simulink model "pmsm_foc_model"  (R2024b)
settings: Solver=ode4  StartTime=0.0  StopTime=.25001  FixedStep=5e-6  RelTol=1e-3
InitFcn:
  | model_dir=fileparts(get_param(bdroot,'FileName')); addpath(fullfile(model_dir,'..','matlab')); addpath(fullfile(model_dir,'..','..','..','build','research_host'));
model workspace (MAT data in the model file):
  cfg.p.Rs = 5.5
  cfg.p.Ld = 0.0007185
  cfg.p.Lq = 0.000905
  cfg.p.psi = 0.00257
  cfg.p.poles = 7
  cfg.p.Vbus = 12
  cfg.p.shunt = 0.02
  cfg.p.gain = 50
  cfg.p.Vref = 3.3
  cfg.p.bits = 12
  cfg.p.ref = 1.65
  cfg.p.lsb = 0.0008056640625
  cfg.p.Ts = 0.001
  cfg.p.fpwm = 20000
  cfg.p.adc_clock = 12000000
  cfg.p.aperture = 6.25e-07
  cfg.p.conversion = 1.66666666667e-06
  cfg.p.bw = 80000
  cfg.p.recovery_tau = 2e-05
  cfg.p.b0 = [0.004 -0.003]
  cfg.p.k = [0.123 0.118]
  cfg.p.kp = 0.5
  cfg.p.ki = 150
  cfg.p.tracking = 200
  cfg.p.ref_limit = 0.04
  cfg.p.mod_limit = 0.0577350269
  cfg.p.seed = 2801
  cfg.dt = 5e-06
  cfg.duration = 0.25
  cfg.reference = 0.04
  cfg.method = "offline_M1"
  cfg.guard = "original"
  cfg.bias_model = "M1"
  cfg.sensor_noise = 0.0008
  cfg.seed = 2801
  cfg.delay = 0.000775
  cfg.omega = 0
  cfg.motion = "locked"
  cfg.J = 2e-05
  cfg.B = 2e-05
  cfg.load = 0
  cfg.adc_phase_s = 0.00025
  cfg.Rfactor = 1
  cfg.Lfactor = 1
  cfg.psifactor = 1
  cfg.bus = 12
  cfg.bias_factor = 1
  cfg.temp_shift = 0
  cfg.esoA = [0.00114141670648  0; 0  1]
  cfg.esoB = [0.181610651508; 0]
  cfg.esoC = [1 1]
  cfg.esoK = [-663.509924553; 0.016548610477]
  cfg.certified = 0
  cfg.error_bound = [0.003; 0.003]
  cfg.fit.model = "M1"
  cfg.fit.coef = {[0.00396479988498; 0.123043689108], [-0.00296998501666; 0.117863719572]}
  cfg.fit.ci95 = {[0.00382515493307  0.00410444483689; 0.122781063704  0.123306314513], [-0.00311154324492  -0.00282842678841; 0.117594560495  0.118132878649]}
  cfg.fit.rank = [2 2]
  cfg.fit.condition = [7.72107695202 7.575631139]
  cfg.noise = [3.05609968406e-05 0.000138698185568 -0.00168675785383 -0.00117877986568 0.000708300191208 0.000612576864667 0.000162588627627 0.000618469759852 0.00109376547218 -0.00161987518611 -0.00119761794175 -0.000644839674806 ... (504 elements, 252x2)]
settings Model: Creator=Administrator  LastModifiedBy=Administrator

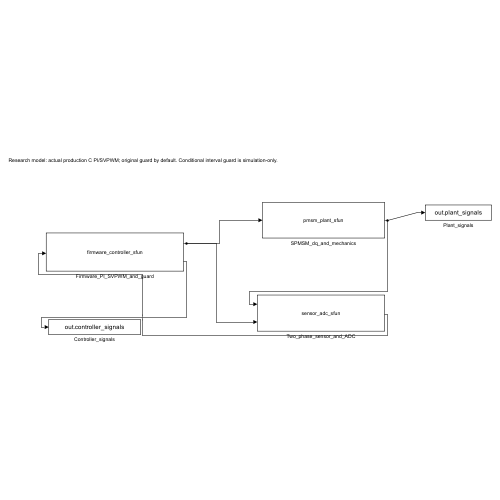
[thumbnail: Simulink's stored preview of the top-level diagram]
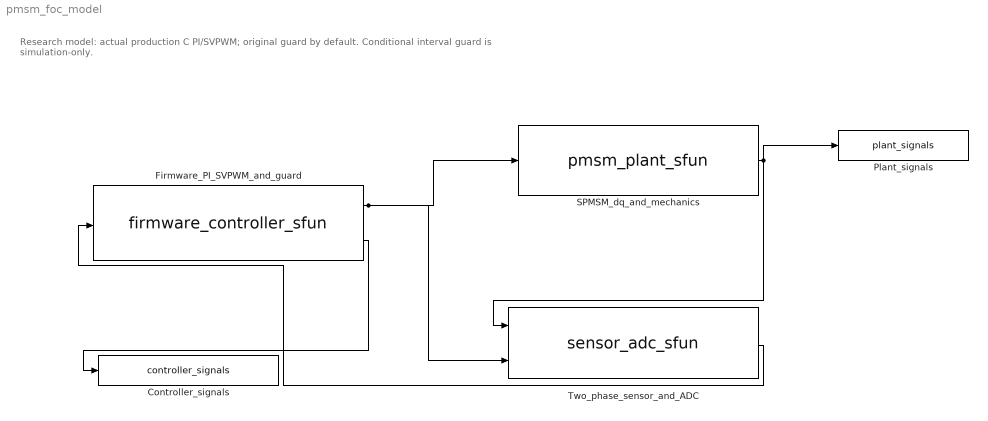
== system pmsm_foc_model ==
  note: Research model: actual production C PI/SVPWM; original guard by default. Conditional interval guard is simulation-only.
  Controller_signals : ToWorkspace  VariableName=controller_signals  SaveFormat=Timeseries  SampleTime=-1
  Firmware_PI_SVPWM_and_guard : M-S-Function  FunctionName=firmware_controller_sfun  Parameters=cfg
  Plant_signals : ToWorkspace  VariableName=plant_signals  SaveFormat=Timeseries  SampleTime=-1
  SPMSM_dq_and_mechanics : M-S-Function  FunctionName=pmsm_plant_sfun  Parameters=cfg
  Two_phase_sensor_and_ADC : M-S-Function  FunctionName=sensor_adc_sfun  Parameters=cfg
  wires:
  Firmware_PI_SVPWM_and_guard/1 -> SPMSM_dq_and_mechanics/1, Two_phase_sensor_and_ADC/2
  SPMSM_dq_and_mechanics/1 -> Two_phase_sensor_and_ADC/1, Plant_signals/1
  Two_phase_sensor_and_ADC/1 -> Firmware_PI_SVPWM_and_guard/1
  Firmware_PI_SVPWM_and_guard/2 -> Controller_signals/1
